simulink model "DIGITAL_WATCH_STAGE3"  (R2026b)
settings: Solver=VariableStepAuto  StopTime=20
libraries: simulink_extras x4
settings Model: Creator=Trealer  LastModifiedBy=Trealer

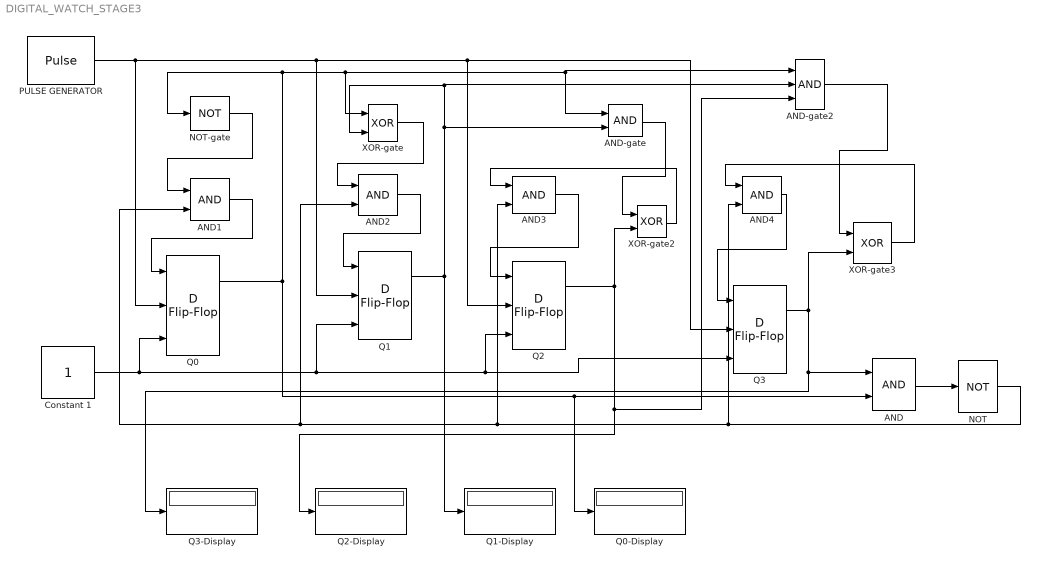
== system DIGITAL_WATCH_STAGE3 ==
  AND{,1..4} (5 alike) : Logic  IconShape=distinctive  AllPortsSameDT=off  OutDataTypeStr=boolean
  AND-gate : Logic  IconShape=distinctive  AllPortsSameDT=off  OutDataTypeStr=boolean
  AND-gate2 : Logic  Inputs=3  IconShape=distinctive  AllPortsSameDT=off  OutDataTypeStr=boolean
  Constant 1 : Constant
  NOT : Logic  Operator=NOT  IconShape=distinctive  AllPortsSameDT=off  OutDataTypeStr=boolean
  NOT-gate : Logic  Operator=NOT  IconShape=distinctive  AllPortsSameDT=off  OutDataTypeStr=boolean
  PULSE GENERATOR : DiscretePulseGenerator  PulseType=Time based  Period=1  PulseWidth=50
  Q{0..3} (4 alike) : simulink_extras/Flip Flops/D Flip-Flop
  Q0-Display : Display
  Q1-Display : Display
  Q2-Display : Display
  Q3-Display : Display
  XOR-gate : Logic  Operator=XOR  IconShape=distinctive  AllPortsSameDT=off  OutDataTypeStr=boolean
  XOR-gate2 : Logic  Operator=XOR  IconShape=distinctive  AllPortsSameDT=off  OutDataTypeStr=boolean
  XOR-gate3 : Logic  Operator=XOR  IconShape=distinctive  AllPortsSameDT=off  OutDataTypeStr=boolean
  wires:
  PULSE GENERATOR/1 -> Q3/2, Q2/2, Q1/2, Q0/2
  Constant 1/1 -> Q3/3, Q2/3, Q1/3, Q0/3
  Q0/1 -> AND-gate/1, AND-gate2/1, XOR-gate/1, NOT-gate/1, Q0-Display/1, AND/2
  Q1/1 -> AND-gate2/2, XOR-gate/2, AND-gate/2, Q1-Display/1
  AND-gate/1 -> XOR-gate2/1
  Q2/1 -> XOR-gate2/2, Q2-Display/1, AND-gate2/3
  AND-gate2/1 -> XOR-gate3/1
  Q3/1 -> XOR-gate3/2, Q3-Display/1, AND/1
  AND/1 -> NOT/1
  NOT-gate/1 -> AND1/1
  XOR-gate/1 -> AND2/1
  XOR-gate2/1 -> AND3/1
  XOR-gate3/1 -> AND4/1
  AND1/1 -> Q0/1
  AND2/1 -> Q1/1
  AND3/1 -> Q2/1
  AND4/1 -> Q3/1
  NOT/1 -> AND4/2, AND3/2, AND1/2, AND2/2
